simulink model "TSPMeA_cycle"  (R2023a)
settings: Solver=VariableStepAuto  StartTime=0.0  StopTime=50E5  FixedStep=1
libraries: nesl_utility x9, fl_lib x8
settings Model: Creator=widana_d  LastModifiedBy=widana_d
settings SolverCC: MaxConsecutiveMinStep=2
settings DataIOCC: SaveFinalState=on  SaveState=on
settings OptimizationCC: ReuseModelBlockBuffer=off
settings ModelReferenceCC: EnableRefExpFcnMdlSchedulingChecks=on
settings SimscapeCC: SimscapeLogType=all  SimscapeLogToSDI=on  SimscapeLogLimitData=off

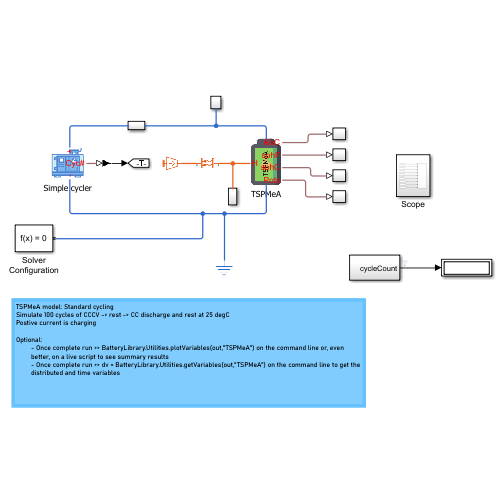
[thumbnail: Simulink's stored preview of the top-level diagram]
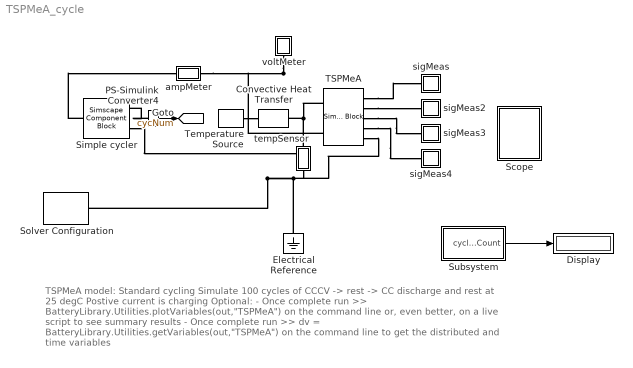
== system TSPMeA_cycle ==
  note: TSPMeA model: Standard cycling
      | Simulate 100 cycles of CCCV -> rest -> CC discharge and rest at 25 degC
      | Postive current is charging
      |
      | Optional:
      | - Once complete run >> BatteryLibrary.Utilities.plotVariables(out,"TSPMeA") on the command line or, even better, on a live script to see summary results
      | - Once complete run >> dv = BatteryLibrary.Utilities.getVariables(out,"TSPMeA") on the command line to get the distributed and time variables
  Convective Heat Transfer : fl_lib/Thermal/Thermal Elements/Convective Heat Transfer  thermal_type=foundation.enum.constant_variable.constant  area=0.0046 m^2  heat_tr_coeff=10 W/(m^2 * K)  min_heat_tr_coeff=1e-3 W/(K*m^2)  T_specify=off  T_priority=None  T=0 K  T_nominal_specify=off  T_nominal_unit=K  T_nominal_value=1  Q_specify=off  Q_priority=None  Q=0 W  Q_nominal_specify=off  Q_nominal_unit=W  Q_nominal_value=1
  Display : Display
  Electrical Reference : fl_lib/Electrical/Electrical Elements/Electrical Reference
  PS-Simulink Converter4 : nesl_utility/PS-Simulink Converter  PhysicalDomain=network_engine_domain  SubClassName=ps_output  LeftPortType=input  RightPortType=output  PseudoPeriodic=off  Frequencies=[]  VectorFormat=1-D array  Unit=inherit  AffineConversion=off
  Scope : Subsystem
  Simple cycler : SimscapeComponentBlock  SourceFile=BatteryLibrary.Utilities.BatteryCycler  ComponentPath=BatteryLibrary.Utilities.BatteryCycler  ComponentVariants="[\"BatteryLibrary.Utilities.BatteryCycler\"]"  ComponentVariantNames="[\"BatteryCycler\"]"  ClassName=BatteryCycler  SchemaVersion=1  Vmax=4.2 V  Vmin=2.5 V  Ic=5/3 A  Ico=0.5 A  Id=-5 A  tRestC=3600 s  tRestD=3600 s
      settings: CopyFcn=simscape.engine.sli.internal.componentblockcallback(gcbh,'COPY')  PreCopyFcn=simscape.engine.sli.internal.componentblockcallback(gcbh,'PRECOPY')  PreDeleteFcn=simscape.engine.sli.internal.componentblockcallback(gcbh,'PREDELETE')  InternalSimscapePortConfiguration="{\"Bottom\":[{\"id\":\"n\",\"label\":\"-\",\"type\":\"foundation.electrical.electrical\"}],\"Left\":[],\"Right\":[{\"id\":\"numCyc\",\"label\":\"Cyc#\",\"type\":\"output\"}],\"Top\":[{\"id\":\"p\",\"label\":\"+\",\"type\":\"foundation.electrical.electrical\"}]}"
      mask Type: A simple battery cycler
  Solver Configuration : nesl_utility/Solver Configuration  PhysicalDomain=network_engine_domain  SubClassName=solver  LeftPortType=input  RightPortType=generic  Tones=[]  Harmonics=[]  SimulateNoise=off  Profile=off  UseLocalSampling=off  EnableSwitchedLinearOptims=on  FrequencyDomain=off  UseCCode=off  RelTol=0.001  AbsTol=1e-06  MinStep=1e-09  ToWorkspace=off  RevertToSquareIcSolve=off  NumHomotopyIterations=100  PhasorMode=off  PhasorModeNumHarmonics=1  ConsistencySolver=NEWTON_FTOL  IndexReductionMethod=DerivativeReplacement  DoDC=off  ResidualTolerance=1e-10  ConsistencyTolSource=GLOBAL  ConsistencyAbsTol=0.001  ConsistencyRelTol=0.001  ConsistencyTolFactor=0.001  UseLocalSolver=off  LocalSolverChoice=NE_BACKWARD_EULER_ADVANCER  ResolveIndetEquations=on  FunctionEvalNumThread=1  LocalSolverSampleTime=0.001  DoFixedCost=off  MaxNonlinIter=3  MaxModeIter=2  ComputeImpulses=off  ImpulseIterations=2  LinearAlgebra=auto  LinearAlgebraNumThread=0  EquationFormulation=NE_TIME_EF  DelaysMemoryBudget=1024  AutomaticFiltering=on  FilteringTimeConstant=0.001  PartitionStorageMethod=AS_NEEDED  PartitionMemoryBudget=1024  PartitionMethod=ROBUST
  Subsystem : Subsystem
  TSPMeA : SimscapeComponentBlock  SourceFile=BatteryLibrary.Models.TSPMeA  ComponentPath=BatteryLibrary.Models.TSPMeA  ComponentVariants="[\"BatteryLibrary.Models.TSPMeA\"]"  ComponentVariantNames="[\"TSPMeA\"]"  ClassName=TSPMeA  SchemaVersion=1  z0=0.5  T0=25 degC  eps_n0=0.3  Lf0=5E-3 um  Cn=4.9 A*hr  DnRef=3.3E-14 m^2/s  DpRef=4E-15 m^2/s  sigma_nRef=215 S/m  sigma_eRef=1.2 S/m  sigma_pRef=0.18 S/m  tr=0.2594  ce0=1000 mol/m^3  cn_max=33133 mol/m^3  cp_max=63104 mol/m^3  sn_max=0.9014  sn_min=0.0279  sp_max=0.9072  sp_min=0.2567  knRef=6.48E-7 A*m^(5/2)/mol^(3/2)  kpRef=3.42E-6 A*m^(5/2)/mol^(3/2)  Cp=110 J/K  Tref=298 K  Ea_kn=10 kJ/mol  Ea_kp=10 kJ/mol  Ea_Dn=8 kJ/mol  Ea_De=8 kJ/mol  Ea_Dp=8 kJ/mol  Ea_sigman=3 kJ/mol  Ea_sigmae=3 kJ/mol  Ea_sigmap=3 kJ/mol  Ea_ksei=50 kJ/mol  Ea_Dsei=10 kJ/mol  Ea_sigmasei=10 kJ/mol  Ea_kLi=2 kJ/mol  kseiRef=1E-11 m/s  DseiRef=2E-21 m^2/s  sigma_seiRef=5E-6 S/m  Msei=0.162 kg/mol  pho_sei=1690 kg/m^3  Usei=0.4 V  csei0=4541 mol/m^3  kLiRef=1E-15 m/s  ULi=0.4 V  MLi=6.94E-3 kg/mol  pho_Li=534 kg/m^3  Ln=85.2 um  Ls=12 um  Lp=75.6 um  Area_p=1027 cm^2  eps_s=0.47  eps_p=0.335  Rn=5.86 um  Rp=5.22 um  an=3.84E5 1/m  ap=3.82E5 1/m
      settings: CopyFcn=simscape.engine.sli.internal.componentblockcallback(gcbh,'COPY')  PreCopyFcn=simscape.engine.sli.internal.componentblockcallback(gcbh,'PRECOPY')  PreDeleteFcn=simscape.engine.sli.internal.componentblockcallback(gcbh,'PREDELETE')  InternalSimscapePortConfiguration="{\"Bottom\":[{\"id\":\"n\",\"label\":\"-\",\"type\":\"foundation.electrical.electrical\"}],\"Left\":[{\"id\":\"Hi\",\"label\":\"H\",\"type\":\"foundation.thermal.thermal\"}],\"Right\":[{\"id\":\"z\",\"label\":\"SoC\",\"type\":\"output\"},{\"id\":\"Lf_bar\",\"label\":\"sohF\",\"type\":\"output\"},{\"id\":\"SoH_Cn\",\"label\":\"sohC\",\"type\":\"output\"},{\"id\":\"pots\",\"label\":\"Pots\",\"type\":\"output\"}],\"Top\":[{\"id\":\"p\",\"label\":\"+\",\"type\":\"foundation.electrical.electrical\"}]}"
      mask Type: TSPMeA
  Temperature Source : fl_lib/Thermal/Thermal Sources/Temperature Source  temperature=25 degC
  ampMeter : Subsystem
  sigMeas : Subsystem
  sigMeas2 : Subsystem
  sigMeas3 : Subsystem
  sigMeas4 : Subsystem
  tempSensor : Subsystem
  voltMeter : Subsystem
  tag scope: cycNum=global
  wires:
  Subsystem/1(cycleCount) -> Display/1
  PS-Simulink Converter4/1 -> [cycNum]
  connections:
  ampMeter/RConn1 -- TSPMeA/LConn2 -- voltMeter/LConn1
  Solver Configuration/RConn1 -- Simple cycler/RConn2 -- TSPMeA/RConn5 -- Electrical Reference/LConn1
  Simple cycler/LConn1 -- ampMeter/LConn1
  TSPMeA/RConn2 -- sigMeas2/LConn1
  TSPMeA/RConn4 -- sigMeas4/LConn1
  TSPMeA/RConn1 -- sigMeas/LConn1
  TSPMeA/RConn3 -- sigMeas3/LConn1
  tempSensor/LConn1 -- TSPMeA/LConn1 -- Convective Heat Transfer/LConn1
  Temperature Source/LConn1 -- Convective Heat Transfer/RConn1
  PS-Simulink Converter4/LConn1 -- Simple cycler/RConn1

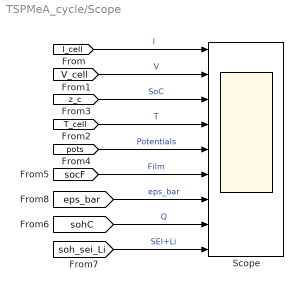
== system TSPMeA_cycle/Scope ==
  Scope : Scope  NumInputPorts=9
  wires:
  [I_cell] -> Scope/1  "I"
  [pots] -> Scope/5  "Potentials"
  [sohC] -> Scope/8  "Q"
  [z_c] -> Scope/3  "SoC"
  [eps_bar] -> Scope/7  "eps_bar"
  [V_cell] -> Scope/2  "V"
  [socF] -> Scope/6  "Film"
  [T_cell] -> Scope/4  "T"
  [soh_sei_Li] -> Scope/9  "SEI+Li"

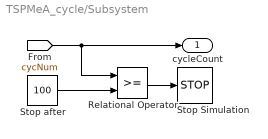
== system TSPMeA_cycle/Subsystem ==
  Relational Operator : RelationalOperator  OutDataTypeStr=boolean  RndMeth=Simplest  InputSameDT=off
  Stop Simulation : Stop
  Stop after : Constant  Value=100
  cycleCount : Outport
  wires:
  Stop after/1 -> Relational Operator/2
  [cycNum] -> Relational Operator/1, cycleCount/1
  Relational Operator/1 -> Stop Simulation/1

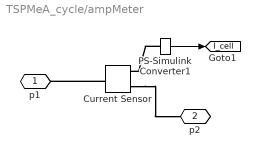
== system TSPMeA_cycle/ampMeter ==
  Current Sensor : fl_lib/Electrical/Electrical Sensors/Current Sensor
  PS-Simulink Converter1 : nesl_utility/PS-Simulink Converter  PhysicalDomain=network_engine_domain  SubClassName=ps_output  LeftPortType=input  RightPortType=output  PseudoPeriodic=off  Frequencies=[]  VectorFormat=1-D array  Unit=inherit  AffineConversion=off
  p1 : PMIOPort  Side=Left
  p2 : PMIOPort  Port=2  Side=Right
  tag scope: I_cell=global
  wires:
  PS-Simulink Converter1/1 -> [I_cell]
  connections:
  Current Sensor/RConn2 -- p2/RConn1
  Current Sensor/LConn1 -- p1/RConn1
  PS-Simulink Converter1/LConn1 -- Current Sensor/RConn1

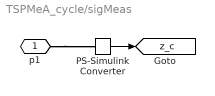
== system TSPMeA_cycle/sigMeas ==
  PS-Simulink Converter : nesl_utility/PS-Simulink Converter  PhysicalDomain=network_engine_domain  SubClassName=ps_output  LeftPortType=input  RightPortType=output  PseudoPeriodic=off  Frequencies=[]  VectorFormat=1-D array  Unit=inherit  AffineConversion=off
  p1 : PMIOPort  Side=Left
  tag scope: z_c=global
  wires:
  PS-Simulink Converter/1 -> [z_c]
  connections:
  p1/RConn1 -- PS-Simulink Converter/LConn1

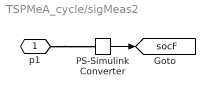
== system TSPMeA_cycle/sigMeas2 ==
  PS-Simulink Converter : nesl_utility/PS-Simulink Converter  PhysicalDomain=network_engine_domain  SubClassName=ps_output  LeftPortType=input  RightPortType=output  PseudoPeriodic=off  Frequencies=[]  VectorFormat=1-D array  Unit=inherit  AffineConversion=off
  p1 : PMIOPort  Side=Left
  tag scope: socF=global
  wires:
  PS-Simulink Converter/1 -> [socF]
  connections:
  p1/RConn1 -- PS-Simulink Converter/LConn1

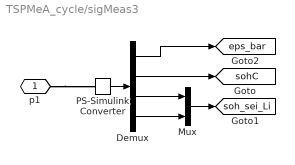
== system TSPMeA_cycle/sigMeas3 ==
  Demux : Demux
  Mux : Mux  Inputs=2
  PS-Simulink Converter : nesl_utility/PS-Simulink Converter  PhysicalDomain=network_engine_domain  SubClassName=ps_output  LeftPortType=input  RightPortType=output  PseudoPeriodic=off  Frequencies=[]  VectorFormat=1-D array  Unit=inherit  AffineConversion=off
  p1 : PMIOPort  Side=Left
  tag scope: eps_bar=global, sohC=global, soh_sei_Li=global
  wires:
  PS-Simulink Converter/1 -> Demux/1
  Mux/1 -> [soh_sei_Li]
  Demux/3 -> Mux/1
  Demux/4 -> Mux/2
  Demux/2 -> [sohC]
  Demux/1 -> [eps_bar]
  connections:
  p1/RConn1 -- PS-Simulink Converter/LConn1

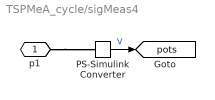
== system TSPMeA_cycle/sigMeas4 ==
  PS-Simulink Converter : nesl_utility/PS-Simulink Converter  PhysicalDomain=network_engine_domain  SubClassName=ps_output  LeftPortType=input  RightPortType=output  PseudoPeriodic=off  Frequencies=[]  VectorFormat=1-D array  Unit=inherit  AffineConversion=off
  p1 : PMIOPort  Side=Left
  tag scope: pots=global
  wires:
  PS-Simulink Converter/1 -> [pots]  "V"
  connections:
  p1/RConn1 -- PS-Simulink Converter/LConn1

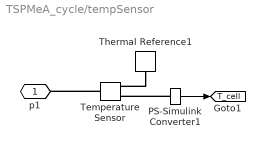
== system TSPMeA_cycle/tempSensor ==
  PS-Simulink Converter1 : nesl_utility/PS-Simulink Converter  PhysicalDomain=network_engine_domain  SubClassName=ps_output  LeftPortType=input  RightPortType=output  PseudoPeriodic=off  Frequencies=[]  VectorFormat=1-D array  Unit=inherit  AffineConversion=off
  Temperature Sensor : fl_lib/Thermal/Thermal Sensors/Temperature Sensor  temperature_measure=foundation.enum.MeasurementReference.difference
  Thermal Reference1 : fl_lib/Thermal/Thermal Elements/Thermal Reference
  p1 : PMIOPort  Side=Left
  tag scope: T_cell=global
  wires:
  PS-Simulink Converter1/1 -> [T_cell]
  connections:
  Temperature Sensor/LConn1 -- p1/RConn1
  PS-Simulink Converter1/LConn1 -- Temperature Sensor/RConn2
  Thermal Reference1/LConn1 -- Temperature Sensor/RConn1

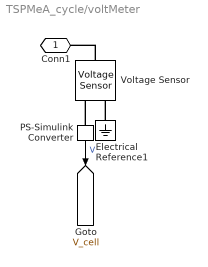
== system TSPMeA_cycle/voltMeter ==
  Electrical Reference1 : fl_lib/Electrical/Electrical Elements/Electrical Reference
  PS-Simulink Converter : nesl_utility/PS-Simulink Converter  PhysicalDomain=network_engine_domain  SubClassName=ps_output  LeftPortType=input  RightPortType=output  PseudoPeriodic=off  Frequencies=[]  VectorFormat=1-D array  Unit=inherit  AffineConversion=off
  Voltage Sensor : fl_lib/Electrical/Electrical Sensors/Voltage Sensor
  Conn1 : PMIOPort  Side=Left
  tag scope: V_cell=global
  wires:
  PS-Simulink Converter/1 -> [V_cell]  "V"
  connections:
  Voltage Sensor/LConn1 -- Conn1/RConn1
  PS-Simulink Converter/LConn1 -- Voltage Sensor/RConn1
  Electrical Reference1/LConn1 -- Voltage Sensor/RConn2
